simulink model "M5_SpeedLoop"  (R2026a)
settings: Solver=ode15s  StopTime=2  MaxStep=0.001
libraries: slpidlib x1
settings Model: Creator=siddh  LastModifiedBy=sjawahar

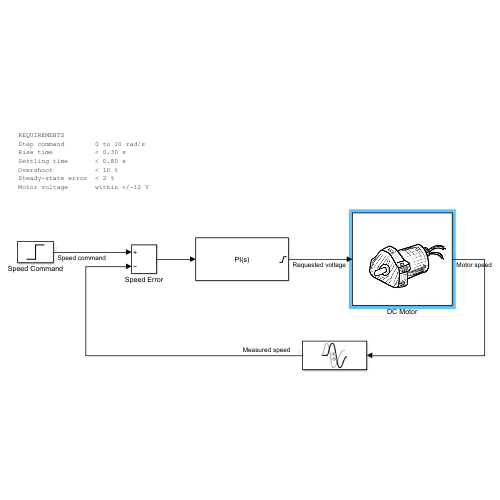
[thumbnail: Simulink's stored preview of the top-level diagram]
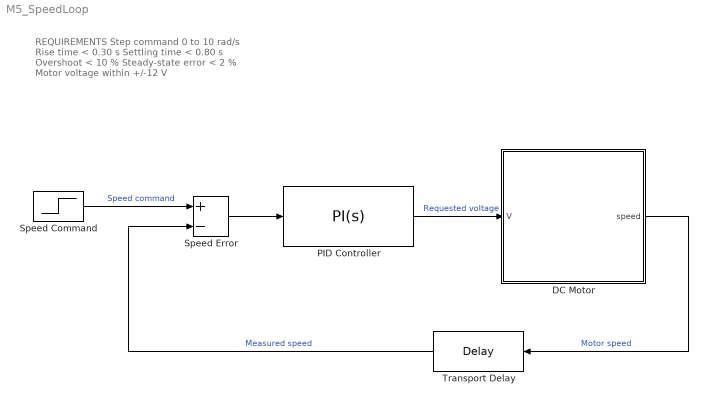
== system M5_SpeedLoop ==
  note: REQUIREMENTS
      | Step command        0 to 10 rad/s
      | Rise time           < 0.30 s
      | Settling time       < 0.80 s
      | Overshoot           < 10 %
      | Steady-state error  < 2 %
      | Motor voltage       within +/-12 V
  DC Motor : Subsystem
      mask Display: image('DC motor.png')
  PID Controller : slpidlib/PID Controller  Controller=PI  Form=Parallel  TimeDomain=Continuous-time  UseExternalTs=off  SampleTime=-1  IntegratorMethod=Forward Euler  FilterMethod=Forward Euler  ControllerParametersSource=internal  P=0.65  I=2.2  UseKiTs=off  D=0  UseExternalDerivativeSource=off  N=100  UseFilter=on  TunerSelectOption=Transfer Function Based (PID Tuner App)  InitialConditionSource=internal  InitialConditionForIntegrator=0  InitialConditionForFilter=0  DifferentiatorICPrevScaledInput=0  ExternalReset=none  TrackingMode=off  Kt=1  LimitOutput=on  SatLimitsSource=internal  UpperSaturationLimit=12  LowerSaturationLimit=-12  LinearizeAsGain=on  AntiWindupMode=clamping  Kb=1  LimitIntegrator=off  UpperIntegratorSaturationLimit=inf  LowerIntegratorSaturationLimit=-inf  POutMin=[]  POutMax=[]  IOutMin=[]  IOutMax=[]  DOutMin=[]  DOutMax=[]  NOutMin=[]  NOutMax=[]  SumOutMin=[]  SumOutMax=[]  SaturationOutMin=[]  SaturationOutMax=[]  PParamMin=[]  PParamMax=[]  IParamMin=[]  IParamMax=[]  DParamMin=[]  DParamMax=[]  NParamMin=[]  NParamMax=[]  KbParamMin=[]  KbParamMax=[]  KtParamMin=[]  KtParamMax=[]  KbOutMin=[]  KbOutMax=[]  KtOutMin=[]  KtOutMax=[]  IntegratorOutMin=[]  IntegratorOutMax=[]  FilterOutMin=[]  FilterOutMax=[]  SumI1OutMin=[]  SumI1OutMax=[]  SumI2OutMin=[]  SumI2OutMax=[]  SumI3OutMin=[]  SumI3OutMax=[]  SumI4OutMin=[]  SumI4OutMax=[]  SumDOutMin=[]  SumDOutMax=[]  DifferentiatorOutMin=[]  DifferentiatorOutMax=[]  FilterDiffOutCoefMin=[]  FilterDiffOutCoefMax=[]  ReciprocalOutMin=[]  ReciprocalOutMax=[]  SumDenOutMin=[]  SumDenOutMax=[]  SumNumOutMin=[]  SumNumOutMax=[]  DivideOutMin=[]  DivideOutMax=[]  UdiffTsProdOutMin=[]  UdiffTsProdOutMax=[]  NTsProdOutMin=[]  NTsProdOutMax=[]  UintegralTsProdOutMin=[]  UintegralTsProdOutMax=[]  UngainTsProdOutMin=[]  UngainTsProdOutMax=[]  ClampingZeroOutDataTypeStr=Inherit: Inherit via back propagation  ClampingZeroOutMin=[]  ClampingZeroOutMax=[]  FilterDenConstantOutDataTypeStr=Inherit: Inherit via back propagation  FilterDenConstantOutMin=[]  FilterDenConstantOutMax=[]  PCopyOutDataTypeStr=Inherit: Inherit via back propagation  PCopyOutMin=[]  PCopyOutMax=[]  NCopyOutDataTypeStr=Inherit: Inherit via back propagation  NCopyOutMin=[]  NCopyOutMax=[]  IntegratorContinuousStateAttributes=''  IntegratorStateMustResolveToSignalObject=off  IntegratorRTWStateStorageClass=Auto  FilterContinuousStateAttributes=''  FilterStateMustResolveToSignalObject=off  FilterRTWStateStorageClass=Auto  ParallelPVariant=InternalParameters  IdealPVariant=Disabled  IVariant=InternalParameters  DVariant=Disabled  IntegratorVariant=Continuous  SatVariant=Enabled  AWVariant=ContClampingParallel  PCopyVariant=Disabled  TRVariant=Disabled  FdbkBlocksVariant=Forward  IdealPFdbkVariant=Disabled  SatFdbkVariant=Disabled  DerivativeFilterVariant=Disabled  NVariant=Disabled  NCopyVariant=Disabled_SignalSpec  FilterICVariant=Disabled  IntegratorICVariant=InternalICs  ExternalResetVariant=Disabled  TRSumVariant=Passthrough  SumFdbkVariant=Disabled  SumVariant=Sum_PI  TsampFilterVariant=InternalTs  TsampNgainVariant=Passthrough  TsampIntegralVariant=Disabled_SignalSpec  ExternalSaturationOutDataTypeStr=Inherit: Same as second input  DerivativeSourceVariant=Disabled  PreIntVariant=InternalPreInt
  Speed Command : Step  Time=0.1  FinalValue=10  SampleTime=0
  Speed Error : Sum  Inputs=+-
  Transport Delay : TransportDelay  DelayTime=0.06  PadeOrder=3
  wires:
  Speed Command/1 -> Speed Error/1  "Speed command"
  Speed Error/1 -> PID Controller/1
  PID Controller/1 -> DC Motor/1(V)  "Requested voltage"
  DC Motor/1(speed) -> Transport Delay/1  "Motor speed"
  Transport Delay/1 -> Speed Error/2  "Measured speed"

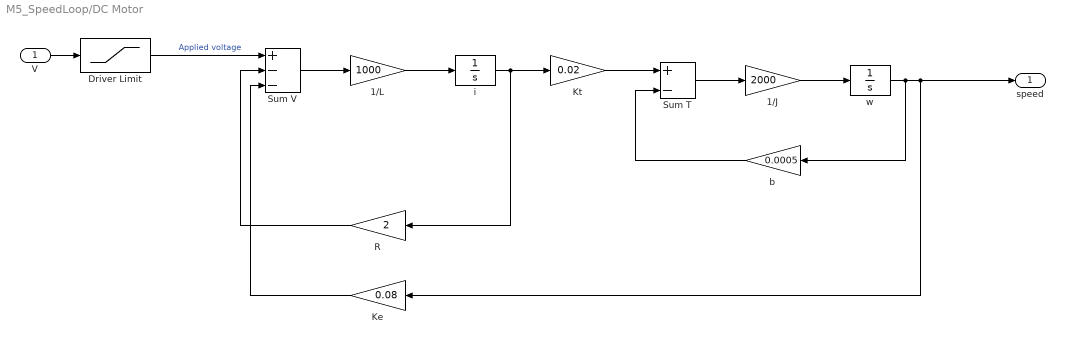
== system M5_SpeedLoop/DC Motor ==
  V : Inport
  1/J : Gain  Gain=2000
  1/L : Gain  Gain=1000
  Driver Limit : Saturate  UpperLimit=12  LowerLimit=-12
  Ke : Gain  Gain=0.08
  Kt : Gain  Gain=0.02
  R : Gain  Gain=2
  Sum T : Sum  Inputs=+-
  Sum V : Sum  Inputs=+--
  b : Gain  Gain=0.0005
  i : Integrator
  w : Integrator
  speed : Outport
  wires:
  V/1 -> Driver Limit/1
  Driver Limit/1 -> Sum V/1  "Applied voltage"
  Sum V/1 -> 1/L/1
  1/L/1 -> i/1
  i/1 -> Kt/1, R/1
  Kt/1 -> Sum T/1
  Sum T/1 -> 1/J/1
  1/J/1 -> w/1
  w/1 -> speed/1, Ke/1, b/1
  b/1 -> Sum T/2
  R/1 -> Sum V/2
  Ke/1 -> Sum V/3
